simulink model "BuckBoost_16V_28V_merged"  (R2021b)
settings: Solver=FixedStepDiscrete  StartTime=0.0  StopTime=p_stop  FixedStep=p_Ts  RelTol=1e-3
model workspace (MAT data in the model file):
  p_Kcurrent = 0.04
  p_Rbleed = 10000
  p_Rload = 14
  p_Rselector = 0.01
  p_Ts = 3.35008375209e-09
  p_boostKi = 80
  p_boostKp = 0.005
  p_buckKi = 40
  p_buckKp = 0.02
  p_iFilterTau = 5e-07
  p_logDecimation = 10
  p_skipBand = 0.03
  p_stop = 0.04
  p_tClose = 0.02005
  p_tOpen = 0.02
  p_vFilterTau = 2e-05
libraries: spsSeriesRLCBranchLib x7, spsCurrentMeasurementLib x5, spsIdealSwitchLib x4, spsVoltageMeasurementLib x3, spsDiodeLib x2, slpidlib x2, simulink x2, spsGroundLib x1, spsDCVoltageSourceLib x1, spspowerguiLib x1
settings Model: Creator=Project contributors  LastModifiedBy=Project contributors
settings DataIOCC: SaveOutput=off  SaveTime=off

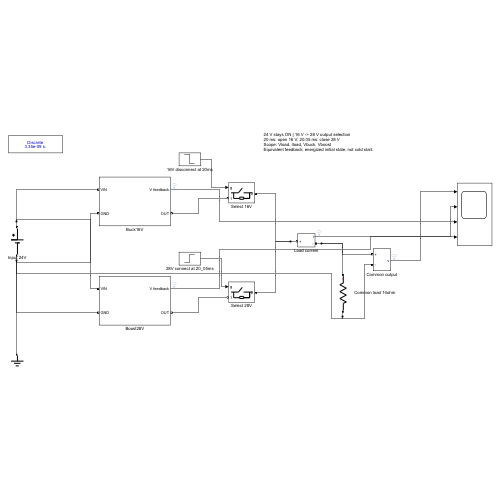
[thumbnail: Simulink's stored preview of the top-level diagram]
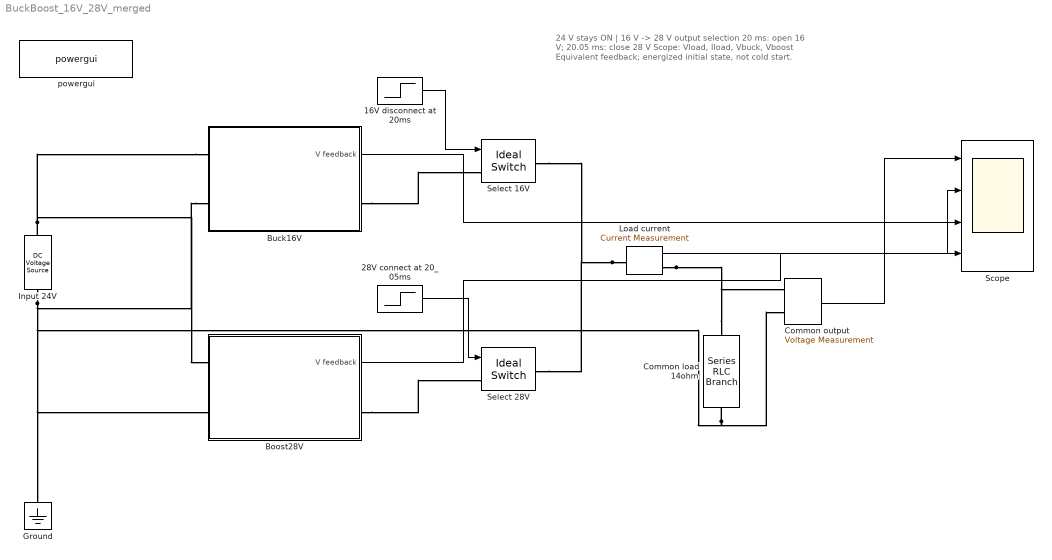
== system BuckBoost_16V_28V_merged ==
  note: 24 V stays ON | 16 V -> 28 V output selection
      | 20 ms: open 16 V; 20.05 ms: close 28 V
      | Scope: Vload, Iload, Vbuck, Vboost
      | Equivalent feedback; energized initial state, not cold start.
  16V disconnect at 20ms : Step  Time=p_tOpen  Before=1  After=0  SampleTime=0
  28V connect at 20_05ms : Step  Time=p_tClose  SampleTime=0
  Boost28V : Subsystem
  Buck16V : Subsystem
  Common load 14ohm : spsSeriesRLCBranchLib/Series RLC Branch  LConnTagsString=__new0  RConnTagsString=__new0  BranchType=R  Resistance=p_Rload  Inductance=1e-3  SetiL0=off  InitialCurrent=0  Capacitance=1e-6  Setx0=off  InitialVoltage=0  Measurements=None
  Common output : spsVoltageMeasurementLib/Voltage Measurement  PhasorSimulation=off  OutputType=Complex  PSBequivalent=0
  Ground : spsGroundLib/Ground  LConnTagsString=a
  Input 24V : spsDCVoltageSourceLib/DC Voltage Source  Amplitude=24  Measurements=None
  Load current : spsCurrentMeasurementLib/Current Measurement  PhasorSimulation=off  OutputType=Complex  PSBequivalent=0
  Scope : Scope  NumInputPorts=4
  Select 16V : spsIdealSwitchLib/Ideal Switch  Ron=p_Rselector  Lon=0  IC=1  Rs=1e6  Cs=inf  Measurements=off
  Select 28V : spsIdealSwitchLib/Ideal Switch  Ron=p_Rselector  Lon=0  IC=0  Rs=1e6  Cs=inf  Measurements=off
  powergui : spspowerguiLib/powergui  Priority=1  SimulationMode=Discrete  SampleTime=p_Ts  frequency=60  Iterations=50  frequencyindice=0  Pbase=100e6  ErrMax=1e-4  UnitsV=kV  UnitsW=MW  buscounter=0  FunctionMessages=off  echomessages=off  EnableUseOfTLC=off  CurrentSourceSwitches=off  DisableSnubberDevices=off  DisableRonSwitches=off  DisableVfSwitches=off  DisplayEquations=off  AutomaticDiscreteSolvers=off  SolverType=Tustin/Backward Euler (TBE)  Interpol=off  ExternalGateDelay=off  methode=off  Ts=100  x0status=blocks  SPID=on  SwTol=0  HookPort=off  NonlinearTolerance=1e-4  nMaxIteration=100  ContinueOnMaxIteration=off  RestoreLinks=warning  ResistiveCurrentMeasurement=off  Frange=[0:2:500]  Ylog=off  Xlog=on  ShowGrid=off  save=off  variable=ZData  structure=0  ZoomFFT=off  StartTime=0.0  cycles=1  DisplayStyle=1  fundamental=60  FreqAxis=off  MaxFrequency=1000  frequencyindicesteady=1  RmsSteady=1  display=off
  wires:
  16V disconnect at 20ms/1 -> Select 16V/1
  28V connect at 20_05ms/1 -> Select 28V/1
  Common output/1 -> Scope/1
  Load current/1 -> Scope/2
  Buck16V/1(V feedback) -> Scope/3
  Boost28V/1(V feedback) -> Scope/4
  connections:
  Buck16V/LConn1 -- Input 24V/RConn1 -- Boost28V/LConn1
  Buck16V/LConn2 -- Input 24V/LConn1 -- Boost28V/LConn2 -- Ground/LConn1 -- Common load 14ohm/RConn1 -- Common output/LConn2
  Buck16V/RConn1 -- Select 16V/LConn1
  Boost28V/RConn1 -- Select 28V/LConn1
  Load current/LConn1 -- Select 16V/RConn1 -- Select 28V/RConn1
  Common load 14ohm/LConn1 -- Load current/RConn1 -- Common output/LConn1

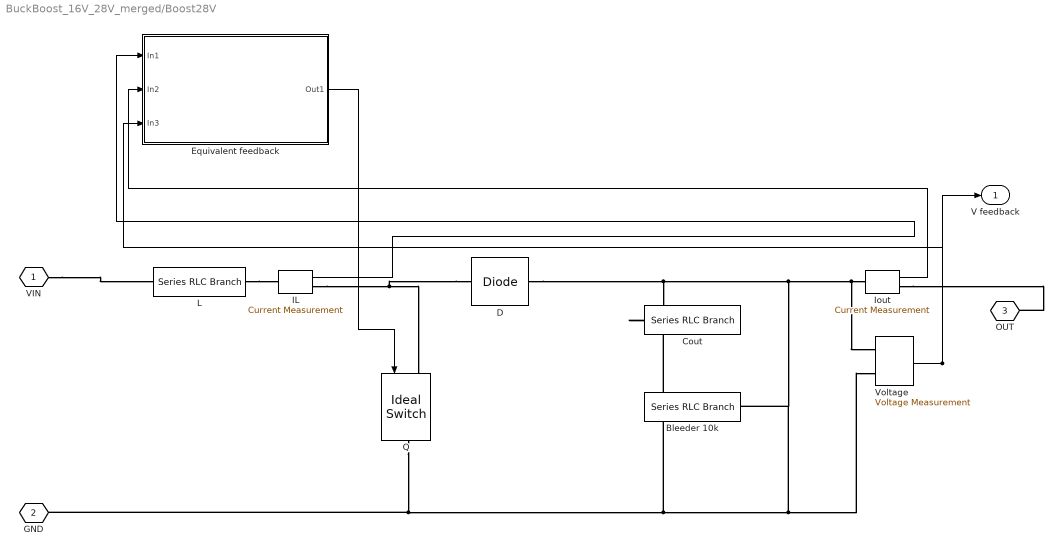
== system BuckBoost_16V_28V_merged/Boost28V ==
  Bleeder 10k : spsSeriesRLCBranchLib/Series RLC Branch  LConnTagsString=__new0  RConnTagsString=__new0  BranchType=R  Resistance=p_Rbleed  Inductance=1e-3  SetiL0=off  InitialCurrent=0  Capacitance=1e-6  Setx0=off  InitialVoltage=0  Measurements=None
  Cout : spsSeriesRLCBranchLib/Series RLC Branch  LConnTagsString=__new0  RConnTagsString=__new0  BranchType=RC  Resistance=0.01  Inductance=1e-3  SetiL0=off  InitialCurrent=0  Capacitance=40e-6  Setx0=on  InitialVoltage=28  Measurements=None
  D : spsDiodeLib/Diode  Ron=0.001  Lon=0  Vf=0.5  IC=0  UseSnubber=0  Rs=500  Cs=250e-9  Measurements=off
  Equivalent feedback : Subsystem
  IL : spsCurrentMeasurementLib/Current Measurement  PhasorSimulation=off  OutputType=Complex  PSBequivalent=0
  Iout : spsCurrentMeasurementLib/Current Measurement  PhasorSimulation=off  OutputType=Complex  PSBequivalent=0
  L : spsSeriesRLCBranchLib/Series RLC Branch  LConnTagsString=__new0  RConnTagsString=__new0  BranchType=RL  Resistance=0.074  Inductance=22e-6  SetiL0=on  InitialCurrent=0  Capacitance=1e-6  Setx0=off  InitialVoltage=0  Measurements=None
  Q : spsIdealSwitchLib/Ideal Switch  Ron=0.06  Lon=0  IC=0  Rs=1e6  Cs=inf  Measurements=off
  Voltage : spsVoltageMeasurementLib/Voltage Measurement  PhasorSimulation=off  OutputType=Complex  PSBequivalent=0
  VIN : PMIOPort  Side=Left
  GND : PMIOPort  Port=2  Side=Left
  OUT : PMIOPort  Port=3  Side=Right
  V feedback : Outport
  wires:
  Voltage/1 -> Equivalent feedback/3(In3), V feedback/1
  IL/1 -> Equivalent feedback/1(In1)
  Iout/1 -> Equivalent feedback/2(In2)
  Equivalent feedback/1(Out1) -> Q/1
  connections:
  VIN/RConn1 -- L/LConn1
  L/RConn1 -- IL/LConn1
  D/LConn1 -- IL/RConn1 -- Q/LConn1
  Q/RConn1 -- Voltage/LConn2 -- Bleeder 10k/RConn1 -- Cout/RConn1 -- GND/RConn1
  Cout/LConn1 -- D/RConn1 -- Voltage/LConn1 -- Iout/LConn1 -- Bleeder 10k/LConn1
  Iout/RConn1 -- OUT/RConn1

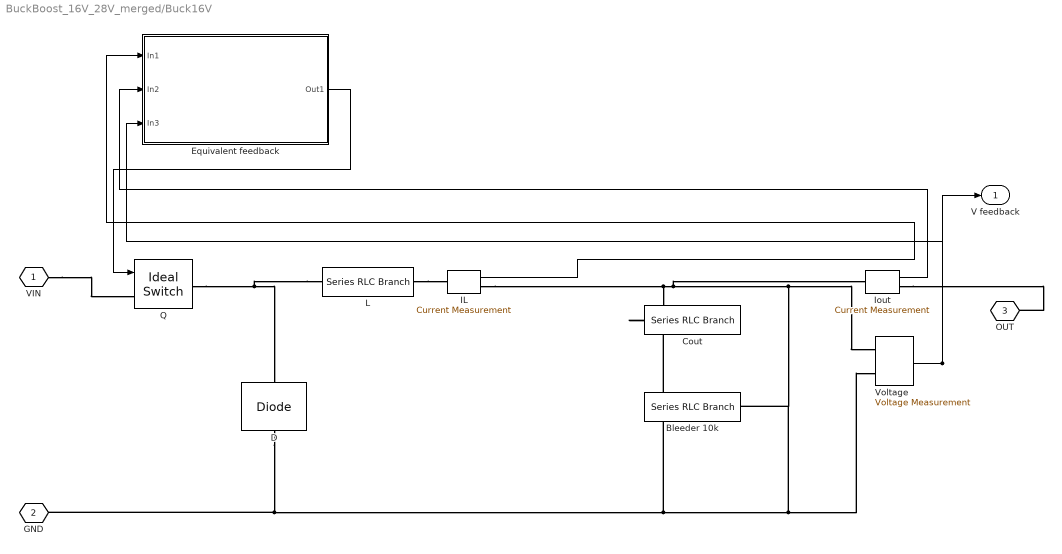
== system BuckBoost_16V_28V_merged/Buck16V ==
  Bleeder 10k : spsSeriesRLCBranchLib/Series RLC Branch  LConnTagsString=__new0  RConnTagsString=__new0  BranchType=R  Resistance=p_Rbleed  Inductance=1e-3  SetiL0=off  InitialCurrent=0  Capacitance=1e-6  Setx0=off  InitialVoltage=0  Measurements=None
  Cout : spsSeriesRLCBranchLib/Series RLC Branch  LConnTagsString=__new0  RConnTagsString=__new0  BranchType=RC  Resistance=0.03  Inductance=1e-3  SetiL0=off  InitialCurrent=0  Capacitance=220e-6  Setx0=on  InitialVoltage=16  Measurements=None
  D : spsDiodeLib/Diode  Ron=0.001  Lon=0  Vf=0.5  IC=0  UseSnubber=0  Rs=500  Cs=250e-9  Measurements=off
  Equivalent feedback : Subsystem
  IL : spsCurrentMeasurementLib/Current Measurement  PhasorSimulation=off  OutputType=Complex  PSBequivalent=0
  Iout : spsCurrentMeasurementLib/Current Measurement  PhasorSimulation=off  OutputType=Complex  PSBequivalent=0
  L : spsSeriesRLCBranchLib/Series RLC Branch  LConnTagsString=__new0  RConnTagsString=__new0  BranchType=RL  Resistance=0.074  Inductance=22e-6  SetiL0=on  InitialCurrent=16/(p_Rload+p_Rselector)+16/p_Rbleed  Capacitance=1e-6  Setx0=off  InitialVoltage=0  Measurements=None
  Q : spsIdealSwitchLib/Ideal Switch  Ron=0.01  Lon=0  IC=0  Rs=1e6  Cs=inf  Measurements=off
  Voltage : spsVoltageMeasurementLib/Voltage Measurement  PhasorSimulation=off  OutputType=Complex  PSBequivalent=0
  VIN : PMIOPort  Side=Left
  GND : PMIOPort  Port=2  Side=Left
  OUT : PMIOPort  Port=3  Side=Right
  V feedback : Outport
  wires:
  Voltage/1 -> Equivalent feedback/3(In3), V feedback/1
  IL/1 -> Equivalent feedback/1(In1)
  Iout/1 -> Equivalent feedback/2(In2)
  Equivalent feedback/1(Out1) -> Q/1
  connections:
  VIN/RConn1 -- Q/LConn1
  L/LConn1 -- Q/RConn1 -- D/RConn1
  D/LConn1 -- Voltage/LConn2 -- Bleeder 10k/RConn1 -- Cout/RConn1 -- GND/RConn1
  L/RConn1 -- IL/LConn1
  Cout/LConn1 -- IL/RConn1 -- Bleeder 10k/LConn1 -- Voltage/LConn1 -- Iout/LConn1
  Iout/RConn1 -- OUT/RConn1

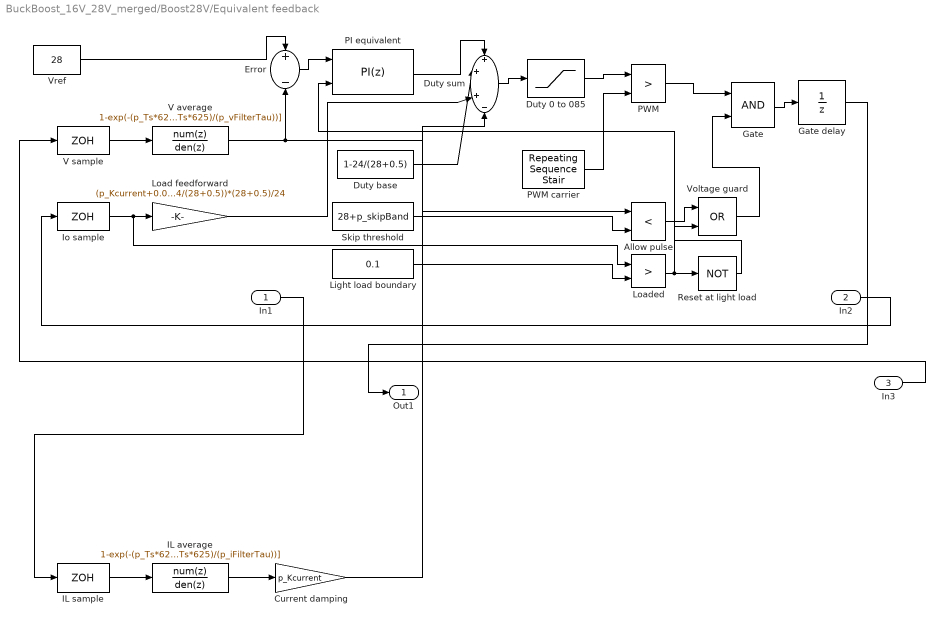
== system BuckBoost_16V_28V_merged/Boost28V/Equivalent feedback ==
  In1 : Inport
  In2 : Inport  Port=2
  In3 : Inport  Port=3
  Allow pulse : RelationalOperator  Operator=<  OutDataTypeStr=boolean  RndMeth=Simplest
  Current damping : Gain  Gain=p_Kcurrent
  Duty 0 to 085 : Saturate  UpperLimit=0.85  LowerLimit=0
  Duty base : Constant  Value=1-24/(28+0.5)
  Duty sum : Sum  Inputs=+++-
  Error : Sum  Inputs=+-
  Gate : Logic  AllPortsSameDT=off  OutDataTypeStr=boolean
  Gate delay : UnitDelay  SampleTime=p_Ts  HasFrameUpgradeWarning=on
  IL average : DiscreteTransferFcn  Numerator=1-exp(-(p_Ts*625)/(p_iFilterTau))  Denominator=[1 -exp(-(p_Ts*625)/(p_iFilterTau))]  InitialStates=(0)/(1-(exp(-(p_Ts*625)/(p_iFilterTau))))  SampleTime=p_Ts*625
  IL sample : ZeroOrderHold  SampleTime=p_Ts*625
  Io sample : ZeroOrderHold  SampleTime=p_Ts*625
  Light load boundary : Constant  Value=0.1
  Load feedforward : Gain  Gain=(p_Kcurrent+0.074/(28+0.5))*(28+0.5)/24
  Loaded : RelationalOperator  Operator=>  OutDataTypeStr=boolean  RndMeth=Simplest
  PI equivalent : slpidlib/PID Controller  Controller=PI  Form=Parallel  TimeDomain=Discrete-time  UseExternalTs=off  SampleTime=p_Ts*625  IntegratorMethod=Forward Euler  FilterMethod=Forward Euler  ControllerParametersSource=internal  P=p_boostKp  I=p_boostKi  D=0  UseFilter=on  N=100  TunerSelectOption=Transfer Function Based (PID Tuner App)  InitialConditionSource=internal  InitialConditionForIntegrator=0  InitialConditionForFilter=0  DifferentiatorICPrevScaledInput=0  ExternalReset=level  TrackingMode=off  Kt=1  LimitOutput=on  SatLimitsSource=internal  UpperSaturationLimit=0.3  LowerSaturationLimit=-0.2  LinearizeAsGain=off  AntiWindupMode=clamping  Kb=1  POutMin=[]  POutMax=[]  IOutMin=[]  IOutMax=[]  DOutMin=[]  DOutMax=[]  NOutMin=[]  NOutMax=[]  SumOutMin=[]  SumOutMax=[]  SaturationOutMin=[]  SaturationOutMax=[]  PParamMin=[]  PParamMax=[]  IParamMin=[]  IParamMax=[]  DParamMin=[]  DParamMax=[]  NParamMin=[]  NParamMax=[]  KbParamMin=[]  KbParamMax=[]  KtParamMin=[]  KtParamMax=[]  KbOutMin=[]  KbOutMax=[]  KtOutMin=[]  KtOutMax=[]  IntegratorOutMin=[]  IntegratorOutMax=[]  FilterOutMin=[]  FilterOutMax=[]  SumI1OutMin=[]  SumI1OutMax=[]  SumI2OutMin=[]  SumI2OutMax=[]  SumI3OutMin=[]  SumI3OutMax=[]  SumI4OutMin=[]  SumI4OutMax=[]  SumDOutMin=[]  SumDOutMax=[]  DifferentiatorOutMin=[]  DifferentiatorOutMax=[]  FilterDiffOutCoefMin=[]  FilterDiffOutCoefMax=[]  ReciprocalOutMin=[]  ReciprocalOutMax=[]  SumDenOutMin=[]  SumDenOutMax=[]  SumNumOutMin=[]  SumNumOutMax=[]  DivideOutMin=[]  DivideOutMax=[]  UdiffTsProdOutMin=[]  UdiffTsProdOutMax=[]  NTsProdOutMin=[]  NTsProdOutMax=[]  UintegralTsProdOutMin=[]  UintegralTsProdOutMax=[]  UngainTsProdOutMin=[]  UngainTsProdOutMax=[]  IntegratorContinuousStateAttributes=''  IntegratorStateMustResolveToSignalObject=off  IntegratorRTWStateStorageClass=Auto  FilterContinuousStateAttributes=''  FilterStateMustResolveToSignalObject=off  FilterRTWStateStorageClass=Auto  ParallelPVariant=InternalParameters  IdealPVariant=Disabled  IVariant=InternalParameters  DVariant=Disabled  IntegratorVariant=Discrete  SatVariant=Enabled  AWVariant=DiscClampingParallel  PCopyVariant=Disabled  TRVariant=Disabled  FdbkBlocksVariant=Forward  IdealPFdbkVariant=Disabled  SatFdbkVariant=Disabled  DerivativeFilterVariant=Disabled  NVariant=Disabled  NCopyVariant=Disabled_SignalSpec  FilterICVariant=Disabled  IntegratorICVariant=InternalICs  ExternalResetVariant=ExternalReset  TRSumVariant=Passthrough  SumFdbkVariant=Disabled  SumVariant=Sum_PI  TsampFilterVariant=InternalTs  TsampNgainVariant=Passthrough  TsampIntegralVariant=Passthrough  ExternalSaturationOutDataTypeStr=Inherit: Same as second input
  PWM : RelationalOperator  Operator=>  OutDataTypeStr=boolean  RndMeth=Simplest
  PWM carrier : simulink/Sources/Repeating Sequence Stair  OutValues=((0:624)+0.5)/625  tsamp=p_Ts  OutMin=[]  OutMax=[]  OutDataTypeStr=double  OutputDataTypeScalingMode=double  OutDataType=fixdt(0,8)  ConRadixGroup=Best Precision: Vector-wise  OutScaling=2^-12
  Reset at light load : Logic  Operator=NOT  AllPortsSameDT=off  OutDataTypeStr=boolean
  Skip threshold : Constant  Value=28+p_skipBand
  V average : DiscreteTransferFcn  Numerator=1-exp(-(p_Ts*625)/(p_vFilterTau))  Denominator=[1 -exp(-(p_Ts*625)/(p_vFilterTau))]  InitialStates=(28)/(1-(exp(-(p_Ts*625)/(p_vFilterTau))))  SampleTime=p_Ts*625
  V sample : ZeroOrderHold  SampleTime=p_Ts*625
  Voltage guard : Logic  Operator=OR  AllPortsSameDT=off  OutDataTypeStr=boolean
  Vref : Constant  Value=28
  Out1 : Outport
  wires:
  V average/1 -> Error/2, Allow pulse/1
  Reset at light load/1 -> PI equivalent/2
  PI equivalent/1 -> Duty sum/1
  Vref/1 -> Error/1
  Duty 0 to 085/1 -> PWM/1
  IL sample/1 -> IL average/1
  Skip threshold/1 -> Allow pulse/2
  Duty base/1 -> Duty sum/2
  Load feedforward/1 -> Duty sum/3
  Io sample/1 -> Load feedforward/1, Loaded/1
  In2/1 -> Io sample/1
  IL average/1 -> Current damping/1
  Error/1 -> PI equivalent/1
  V sample/1 -> V average/1
  Light load boundary/1 -> Loaded/2
  Loaded/1 -> Reset at light load/1, Voltage guard/2
  PWM/1 -> Gate/1
  Current damping/1 -> Duty sum/4
  Gate/1 -> Gate delay/1
  Voltage guard/1 -> Gate/2
  Gate delay/1 -> Out1/1
  PWM carrier/1 -> PWM/2
  Duty sum/1 -> Duty 0 to 085/1
  Allow pulse/1 -> Voltage guard/1
  In1/1 -> IL sample/1
  In3/1 -> V sample/1

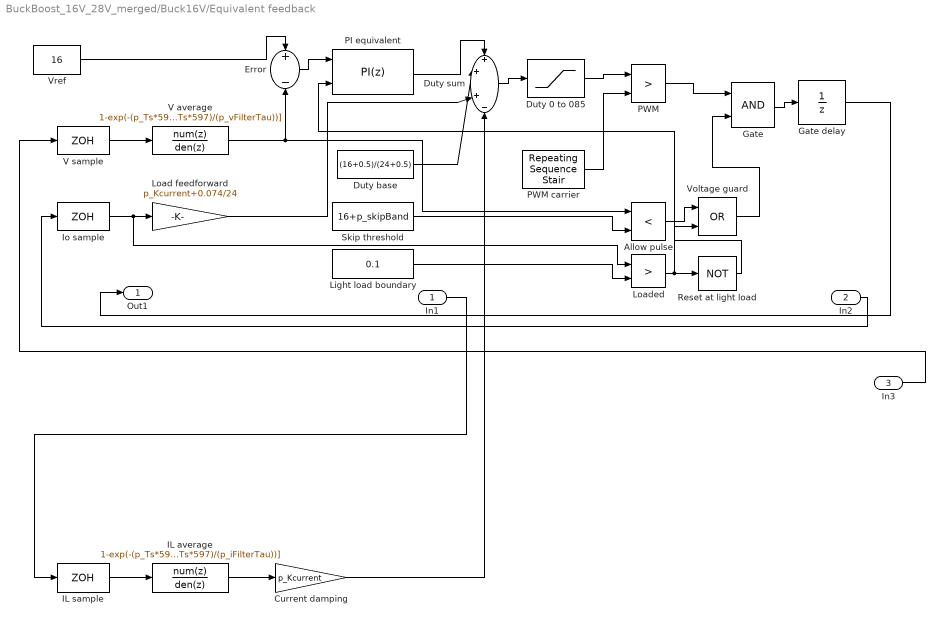
== system BuckBoost_16V_28V_merged/Buck16V/Equivalent feedback ==
  In1 : Inport
  In2 : Inport  Port=2
  In3 : Inport  Port=3
  Allow pulse : RelationalOperator  Operator=<  OutDataTypeStr=boolean  RndMeth=Simplest
  Current damping : Gain  Gain=p_Kcurrent
  Duty 0 to 085 : Saturate  UpperLimit=0.85  LowerLimit=0
  Duty base : Constant  Value=(16+0.5)/(24+0.5)
  Duty sum : Sum  Inputs=+++-
  Error : Sum  Inputs=+-
  Gate : Logic  AllPortsSameDT=off  OutDataTypeStr=boolean
  Gate delay : UnitDelay  SampleTime=p_Ts  HasFrameUpgradeWarning=on
  IL average : DiscreteTransferFcn  Numerator=1-exp(-(p_Ts*597)/(p_iFilterTau))  Denominator=[1 -exp(-(p_Ts*597)/(p_iFilterTau))]  InitialStates=(16/(p_Rload+p_Rselector)+16/p_Rbleed)/(1-(exp(-(p_Ts*597)/(p_iFilterTau))))  SampleTime=p_Ts*597
  IL sample : ZeroOrderHold  SampleTime=p_Ts*597
  Io sample : ZeroOrderHold  SampleTime=p_Ts*597
  Light load boundary : Constant  Value=0.1
  Load feedforward : Gain  Gain=p_Kcurrent+0.074/24
  Loaded : RelationalOperator  Operator=>  OutDataTypeStr=boolean  RndMeth=Simplest
  PI equivalent : slpidlib/PID Controller  Controller=PI  Form=Parallel  TimeDomain=Discrete-time  UseExternalTs=off  SampleTime=p_Ts*597  IntegratorMethod=Forward Euler  FilterMethod=Forward Euler  ControllerParametersSource=internal  P=p_buckKp  I=p_buckKi  D=0  UseFilter=on  N=100  TunerSelectOption=Transfer Function Based (PID Tuner App)  InitialConditionSource=internal  InitialConditionForIntegrator=0  InitialConditionForFilter=0  DifferentiatorICPrevScaledInput=0  ExternalReset=level  TrackingMode=off  Kt=1  LimitOutput=on  SatLimitsSource=internal  UpperSaturationLimit=0.3  LowerSaturationLimit=-0.2  LinearizeAsGain=off  AntiWindupMode=clamping  Kb=1  POutMin=[]  POutMax=[]  IOutMin=[]  IOutMax=[]  DOutMin=[]  DOutMax=[]  NOutMin=[]  NOutMax=[]  SumOutMin=[]  SumOutMax=[]  SaturationOutMin=[]  SaturationOutMax=[]  PParamMin=[]  PParamMax=[]  IParamMin=[]  IParamMax=[]  DParamMin=[]  DParamMax=[]  NParamMin=[]  NParamMax=[]  KbParamMin=[]  KbParamMax=[]  KtParamMin=[]  KtParamMax=[]  KbOutMin=[]  KbOutMax=[]  KtOutMin=[]  KtOutMax=[]  IntegratorOutMin=[]  IntegratorOutMax=[]  FilterOutMin=[]  FilterOutMax=[]  SumI1OutMin=[]  SumI1OutMax=[]  SumI2OutMin=[]  SumI2OutMax=[]  SumI3OutMin=[]  SumI3OutMax=[]  SumI4OutMin=[]  SumI4OutMax=[]  SumDOutMin=[]  SumDOutMax=[]  DifferentiatorOutMin=[]  DifferentiatorOutMax=[]  FilterDiffOutCoefMin=[]  FilterDiffOutCoefMax=[]  ReciprocalOutMin=[]  ReciprocalOutMax=[]  SumDenOutMin=[]  SumDenOutMax=[]  SumNumOutMin=[]  SumNumOutMax=[]  DivideOutMin=[]  DivideOutMax=[]  UdiffTsProdOutMin=[]  UdiffTsProdOutMax=[]  NTsProdOutMin=[]  NTsProdOutMax=[]  UintegralTsProdOutMin=[]  UintegralTsProdOutMax=[]  UngainTsProdOutMin=[]  UngainTsProdOutMax=[]  IntegratorContinuousStateAttributes=''  IntegratorStateMustResolveToSignalObject=off  IntegratorRTWStateStorageClass=Auto  FilterContinuousStateAttributes=''  FilterStateMustResolveToSignalObject=off  FilterRTWStateStorageClass=Auto  ParallelPVariant=InternalParameters  IdealPVariant=Disabled  IVariant=InternalParameters  DVariant=Disabled  IntegratorVariant=Discrete  SatVariant=Enabled  AWVariant=DiscClampingParallel  PCopyVariant=Disabled  TRVariant=Disabled  FdbkBlocksVariant=Forward  IdealPFdbkVariant=Disabled  SatFdbkVariant=Disabled  DerivativeFilterVariant=Disabled  NVariant=Disabled  NCopyVariant=Disabled_SignalSpec  FilterICVariant=Disabled  IntegratorICVariant=InternalICs  ExternalResetVariant=ExternalReset  TRSumVariant=Passthrough  SumFdbkVariant=Disabled  SumVariant=Sum_PI  TsampFilterVariant=InternalTs  TsampNgainVariant=Passthrough  TsampIntegralVariant=Passthrough  ExternalSaturationOutDataTypeStr=Inherit: Same as second input
  PWM : RelationalOperator  Operator=>  OutDataTypeStr=boolean  RndMeth=Simplest
  PWM carrier : simulink/Sources/Repeating Sequence Stair  OutValues=((0:596)+0.5)/597  tsamp=p_Ts  OutMin=[]  OutMax=[]  OutDataTypeStr=double  OutputDataTypeScalingMode=double  OutDataType=fixdt(0,8)  ConRadixGroup=Best Precision: Vector-wise  OutScaling=2^-12
  Reset at light load : Logic  Operator=NOT  AllPortsSameDT=off  OutDataTypeStr=boolean
  Skip threshold : Constant  Value=16+p_skipBand
  V average : DiscreteTransferFcn  Numerator=1-exp(-(p_Ts*597)/(p_vFilterTau))  Denominator=[1 -exp(-(p_Ts*597)/(p_vFilterTau))]  InitialStates=(16)/(1-(exp(-(p_Ts*597)/(p_vFilterTau))))  SampleTime=p_Ts*597
  V sample : ZeroOrderHold  SampleTime=p_Ts*597
  Voltage guard : Logic  Operator=OR  AllPortsSameDT=off  OutDataTypeStr=boolean
  Vref : Constant  Value=16
  Out1 : Outport
  wires:
  V average/1 -> Error/2, Allow pulse/1
  V sample/1 -> V average/1
  Reset at light load/1 -> PI equivalent/2
  Error/1 -> PI equivalent/1
  Light load boundary/1 -> Loaded/2
  Loaded/1 -> Reset at light load/1, Voltage guard/2
  Vref/1 -> Error/1
  Load feedforward/1 -> Duty sum/3
  Skip threshold/1 -> Allow pulse/2
  Voltage guard/1 -> Gate/2
  Gate/1 -> Gate delay/1
  Gate delay/1 -> Out1/1
  Duty base/1 -> Duty sum/2
  Io sample/1 -> Load feedforward/1, Loaded/1
  In2/1 -> Io sample/1
  PWM carrier/1 -> PWM/2
  Duty sum/1 -> Duty 0 to 085/1
  Duty 0 to 085/1 -> PWM/1
  In3/1 -> V sample/1
  IL average/1 -> Current damping/1
  Current damping/1 -> Duty sum/4
  PI equivalent/1 -> Duty sum/1
  Allow pulse/1 -> Voltage guard/1
  IL sample/1 -> IL average/1
  PWM/1 -> Gate/1
  In1/1 -> IL sample/1
